simulink model "override_n_feedfw_feedbk_ctrl"  (R2024b)
settings: Solver=VariableStepAuto  StartTime=0.0  StopTime=90  RelTol=1e-3
values from neighbouring files (symbols this model uses):
  accel_limit_fuel = [500 1200 1800 2200 2500 2600 2700]    [datas.m]
  actual_rpm_pts = [40 50 60 70 80 90 100]    [datas.m]
  altitude_ft = [0 10000 20000 30000 40000]    [datas.m]
  decel_limit_fuel = [180 180 180 180 180 180 180]    [datas.m]
  delta_rpm_pts = [0 10 20 30 40 50 60]    [datas.m]
  steady_state_fuel = [200 300 450 650 900 1300 1800]    [datas.m]
  throttle_pct = [0 10 20 30 40 50 60 70 80 90 100]    [datas.m]
libraries: slpidlib x1
settings Model: Creator=emrekarausta  LastModifiedBy=emrekarausta

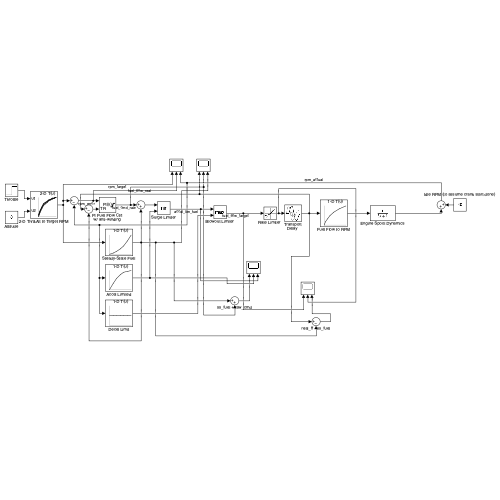
[thumbnail: Simulink's stored preview of the top-level diagram]
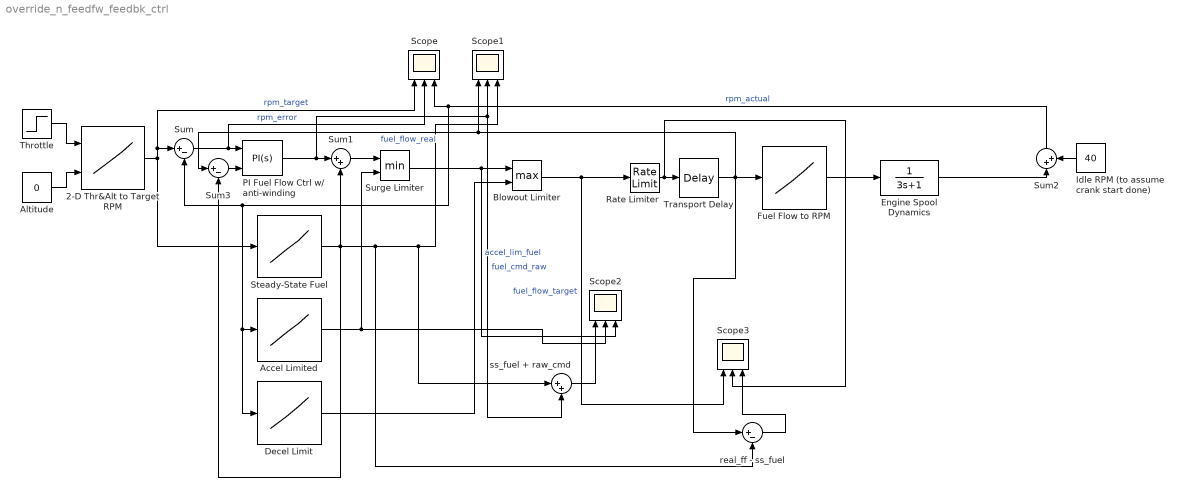
== system override_n_feedfw_feedbk_ctrl ==
  2-D Thr&Alt to Target RPM : Lookup_n-D  BreakpointsForDimension1=throttle_pct  BreakpointsForDimension2=altitude_ft  Table=target_rpm_map'  InternalRulePriority=Speed  RndMeth=Simplest
      settings: InputPortMap=u0,u1
  Accel Limited : Lookup_n-D  NumberOfTableDimensions=1  BreakpointsForDimension1=actual_rpm_pts  Table=accel_limit_fuel  ExtrapMethod=Clip  InternalRulePriority=Speed  RndMeth=Simplest
  Altitude : Constant  Value=0
  Blowout Limiter : MinMax  Function=max  Inputs=2
  Decel Limit : Lookup_n-D  NumberOfTableDimensions=1  BreakpointsForDimension1=actual_rpm_pts  Table=decel_limit_fuel  ExtrapMethod=Clip  InternalRulePriority=Speed  RndMeth=Simplest
  Engine Spool Dynamics : TransferFcn  Denominator=[3 1]
  Fuel Flow to RPM : Lookup_n-D  NumberOfTableDimensions=1  BreakpointsForDimension1=steady_state_fuel  Table=delta_rpm_pts  ExtrapMethod=Clip  InternalRulePriority=Speed  RndMeth=Simplest
  Idle RPM (to assume crank start done) : Constant  Value=40
  PI Fuel Flow Ctrl w/ anti-winding : slpidlib/PID Controller  Controller=PI  Form=Parallel  TimeDomain=Continuous-time  UseExternalTs=off  SampleTime=-1  IntegratorMethod=Forward Euler  FilterMethod=Forward Euler  ControllerParametersSource=internal  P=10.45  I=3.45  UseKiTs=off  D=0  UseExternalDerivativeSource=off  N=100  UseFilter=on  TunerSelectOption=Transfer Function Based (PID Tuner App)  InitialConditionSource=internal  InitialConditionForIntegrator=0  InitialConditionForFilter=0  DifferentiatorICPrevScaledInput=0  ExternalReset=none  TrackingMode=on  Kt=1  LimitOutput=on  SatLimitsSource=internal  UpperSaturationLimit=5000  LowerSaturationLimit=-500  LinearizeAsGain=on  AntiWindupMode=clamping  Kb=1  LimitIntegrator=off  UpperIntegratorSaturationLimit=inf  LowerIntegratorSaturationLimit=-inf  POutMin=[]  POutMax=[]  IOutMin=[]  IOutMax=[]  DOutMin=[]  DOutMax=[]  NOutMin=[]  NOutMax=[]  SumOutMin=[]  SumOutMax=[]  SaturationOutMin=[]  SaturationOutMax=[]  PParamMin=[]  PParamMax=[]  IParamMin=[]  IParamMax=[]  DParamMin=[]  DParamMax=[]  NParamMin=[]  NParamMax=[]  KbParamMin=[]  KbParamMax=[]  KtParamMin=[]  KtParamMax=[]  KbOutMin=[]  KbOutMax=[]  KtOutMin=[]  KtOutMax=[]  IntegratorOutMin=[]  IntegratorOutMax=[]  FilterOutMin=[]  FilterOutMax=[]  SumI1OutMin=[]  SumI1OutMax=[]  SumI2OutMin=[]  SumI2OutMax=[]  SumI3OutMin=[]  SumI3OutMax=[]  SumI4OutMin=[]  SumI4OutMax=[]  SumDOutMin=[]  SumDOutMax=[]  DifferentiatorOutMin=[]  DifferentiatorOutMax=[]  FilterDiffOutCoefMin=[]  FilterDiffOutCoefMax=[]  ReciprocalOutMin=[]  ReciprocalOutMax=[]  SumDenOutMin=[]  SumDenOutMax=[]  SumNumOutMin=[]  SumNumOutMax=[]  DivideOutMin=[]  DivideOutMax=[]  UdiffTsProdOutMin=[]  UdiffTsProdOutMax=[]  NTsProdOutMin=[]  NTsProdOutMax=[]  UintegralTsProdOutMin=[]  UintegralTsProdOutMax=[]  UngainTsProdOutMin=[]  UngainTsProdOutMax=[]  ClampingZeroOutDataTypeStr=Inherit: Inherit via back propagation  ClampingZeroOutMin=[]  ClampingZeroOutMax=[]  FilterDenConstantOutDataTypeStr=Inherit: Inherit via back propagation  FilterDenConstantOutMin=[]  FilterDenConstantOutMax=[]  PCopyOutDataTypeStr=Inherit: Inherit via back propagation  PCopyOutMin=[]  PCopyOutMax=[]  NCopyOutDataTypeStr=Inherit: Inherit via back propagation  NCopyOutMin=[]  NCopyOutMax=[]  IntegratorContinuousStateAttributes=''  IntegratorStateMustResolveToSignalObject=off  IntegratorRTWStateStorageClass=Auto  FilterContinuousStateAttributes=''  FilterStateMustResolveToSignalObject=off  FilterRTWStateStorageClass=Auto  ParallelPVariant=InternalParameters  IdealPVariant=Disabled  IVariant=InternalParameters  DVariant=Disabled  IntegratorVariant=Continuous  SatVariant=Enabled  AWVariant=ContClampingParallel  PCopyVariant=Disabled  TRVariant=Enabled  FdbkBlocksVariant=Forward  IdealPFdbkVariant=Disabled  SatFdbkVariant=Disabled  DerivativeFilterVariant=Disabled  NVariant=Disabled  NCopyVariant=Disabled_SignalSpec  FilterICVariant=Disabled  IntegratorICVariant=InternalICs  ExternalResetVariant=Disabled  TRSumVariant=TrackingMode  SumFdbkVariant=Disabled  SumVariant=Sum_PI  TsampFilterVariant=InternalTs  TsampNgainVariant=Passthrough  TsampIntegralVariant=Disabled_SignalSpec  ExternalSaturationOutDataTypeStr=Inherit: Same as second input  DerivativeSourceVariant=Disabled  PreIntVariant=InternalPreInt
  "Rate Limiter " : RateLimiter  RisingSlewLimit=3000  FallingSlewLimit=-3000  SampleTimeMode=inherited
  Scope{,1..3} (4 alike) : Scope  NumInputPorts=3
  Steady-State Fuel : Lookup_n-D  NumberOfTableDimensions=1  BreakpointsForDimension1=actual_rpm_pts  Table=steady_state_fuel  ExtrapMethod=Clip  InternalRulePriority=Speed  RndMeth=Simplest
  Sum : Sum  Inputs=|+-
  Sum1 : Sum  Inputs=|++
  Sum2 : Sum  Inputs=|++
  Sum3 : Sum  Inputs=|+-
  Surge Limiter : MinMax  Inputs=2
  Throttle : Step  Time=60  Before=25  After=30  SampleTime=0
  "Transport Delay " : TransportDelay  DelayTime=0.1
  real_ff - ss_fuel : Sum  Inputs=|+-
  ss_fuel + raw_cmd : Sum  Inputs=|++
  wires:
  Throttle/1 -> 2-D Thr&Alt to Target RPM/1
  Altitude/1 -> 2-D Thr&Alt to Target RPM/2
  2-D Thr&Alt to Target RPM/1 -> Sum/1, Scope/1, Steady-State Fuel/1  "rpm_target"
  Sum/1 -> Scope/2, PI Fuel Flow Ctrl w/ anti-winding/1  "rpm_error"
  Accel Limited/1 -> Scope2/2, Surge Limiter/2
  Surge Limiter/1 -> Blowout Limiter/1, Scope2/3  "accel_lim_fuel"
  Decel Limit/1 -> Blowout Limiter/2
  PI Fuel Flow Ctrl w/ anti-winding/1 -> ss_fuel + raw_cmd/2, Scope1/2, Sum1/1  "fuel_cmd_raw"
  Sum1/1 -> Surge Limiter/1
  Steady-State Fuel/1 -> real_ff - ss_fuel/2, ss_fuel + raw_cmd/1, Scope1/3, Sum3/2, Sum1/2
  Blowout Limiter/1 -> "Rate Limiter "/1, Scope3/1  "fuel_flow_target"
  "Rate Limiter "/1 -> Scope3/2, "Transport Delay "/1
  "Transport Delay "/1 -> real_ff - ss_fuel/1, Scope1/1, Sum3/1, Fuel Flow to RPM/1  "fuel_flow_real"
  Fuel Flow to RPM/1 -> Engine Spool Dynamics/1
  Idle RPM (to assume crank start done)/1 -> Sum2/2
  Engine Spool Dynamics/1 -> Sum2/1
  Sum2/1 -> Decel Limit/1, Accel Limited/1, Sum/2, Scope/3  "rpm_actual"
  Sum3/1 -> PI Fuel Flow Ctrl w/ anti-winding/2
  ss_fuel + raw_cmd/1 -> Scope2/1
  real_ff - ss_fuel/1 -> Scope3/3
